simulink model "FMS"  (R2018b)
settings: configuration reference "fms_config" (kept outside this file)
values from neighbouring files (symbols this model uses):
  FMS_EXPORT = Simulink.Parameter(FMS_EXPORT_VALUE)    [fms_model_init.m]
  FMS_PARAM = Simulink.Parameter(FMS_PARAM_VALUE)    [fms_model_init.m]
undefined symbols (not defined in the file or in its folder): actuator_cmd, ax_cmd, ay_cmd, az_cmd, cmd_mask, ControlMode, ctrl_mode, DiscIntNeverNeededParam, ext_state, FMS_Cmd, FMS_CONST, home, mode, p_cmd, phi_cmd, PilotMode, psi_rate_cmd, q_cmd, r_cmd, reset, state, status, theta_cmd, throttle_cmd, timestamp, u_cmd, v_cmd, VehicleState, VehicleStatus, VTOLState, w_cmd, wp_consume, wp_current
libraries: simulink x141, FMT_Model_Lib x120, hdlsllib x13
(part 9 of 12)

== system FMS/FMS Commander/Commander/Arm/MC_Mode/Auto/Offboard/Heading_Command/Heading_Control/Error/psi_err_saturation ==
  psi_err_in : Inport
  Abs : Abs
  Compare To Constant : simulink/Logic and Bit Operations/Compare To Constant  relop=>  const=pi  OutDataTypeStr=boolean
  Constant : Constant  Value=2*pi  OutDataTypeStr=single
  Multiply : Product
  Sign : Signum
  Subtract : Sum  Inputs=-+
  Switch : Switch  Criteria=u2 > Threshold
  psi_err_rad : Outport
  wires:
  Multiply/1 -> Switch/1
  Sign/1 -> Multiply/2
  Subtract/1 -> Multiply/1
  Constant/1 -> Subtract/1
  Switch/1 -> psi_err_rad/1
  Compare To Constant/1 -> Switch/2
  Abs/1 -> Compare To Constant/1, Subtract/2
  psi_err_in/1 -> Abs/1, Switch/3, Sign/1

== system FMS/FMS Commander/Commander/Arm/MC_Mode/Auto/Offboard/Velocity_Command/Position_Control/Position_Command/Command_Mask ==
  FMS_In : Inport
  Bus Selector3 : BusSelector  OutputSignals=Auto_Cmd.cmd_mask
  Compare To Zero : simulink/Logic and Bit Operations/Compare To Zero  relop=>  OutDataTypeStr=boolean
  Mux3 : Mux  Inputs=3
  alt_cmd valid : simulink/Logic and Bit Operations/Bitwise Operator  logicop=AND  UseBitMask=on  BitMask=bin2dec('1000000000000')  BitMaskRealWorld=Stored Integer
  lat_cmd valid : simulink/Logic and Bit Operations/Bitwise Operator  logicop=AND  UseBitMask=on  BitMask=bin2dec('10000000000')  BitMaskRealWorld=Stored Integer
  lon_cmd valid : simulink/Logic and Bit Operations/Bitwise Operator  logicop=AND  UseBitMask=on  BitMask=bin2dec('100000000000')  BitMaskRealWorld=Stored Integer
  global_cmd_valid : Outport
  wires:
  Bus Selector3/1 -> alt_cmd valid/1, lat_cmd valid/1, lon_cmd valid/1  "<cmd_mask>"
  lat_cmd valid/1 -> Mux3/1
  FMS_In/1 -> Bus Selector3/1
  Mux3/1 -> Compare To Zero/1
  lon_cmd valid/1 -> Mux3/2
  alt_cmd valid/1 -> Mux3/3
  Compare To Zero/1 -> global_cmd_valid/1

== system FMS/FMS Commander/Commander/Arm/MC_Mode/Auto/Offboard/Velocity_Command/Position_Control/Position_Command/Global_Position_Command ==
  FMS_In : Inport
  Bus Selector1 : BusSelector  OutputSignals=Auto_Cmd.lat_cmd,Auto_Cmd.lon_cmd,Auto_Cmd.alt_cmd
  Bus Selector2 : BusSelector  OutputSignals=INS_Out.lat_0,INS_Out.lon_0,INS_Out.alt_0
  Constant : Constant  Value=0
  Data Type Conversion : DataTypeConversion  OutDataTypeStr=double
  Data Type Conversion1 : DataTypeConversion  OutDataTypeStr=single
  Gain : Gain  Gain=1e-7  OutDataTypeStr=double
  Gain1 : Gain  Gain=1e-7  OutDataTypeStr=double
  Gain2 : Gain  Gain=-1
  LLA2FLAT : FMT_Model_Lib/Transformation/LLA2FLAT
      settings: SourceProductName=FMT Toolbox
  Mux : Mux  Inputs=3
  Mux1 : Mux  Inputs=2
  rad2deg : Gain  Gain=180/pi  OutDataTypeStr=double
  pos_cmd_O : Outport
  wires:
  Bus Selector1/3 -> Data Type Conversion/1  "<alt_cmd>"
  Gain/1 -> Mux/1
  Mux1/1 -> rad2deg/1
  Bus Selector1/1 -> Gain/1  "<lat_cmd>"
  FMS_In/1 -> Bus Selector2/1, Bus Selector1/1
  rad2deg/1 -> LLA2FLAT/2
  Gain1/1 -> Mux/2
  Bus Selector1/2 -> Gain1/1  "<lon_cmd>"
  Mux/1 -> LLA2FLAT/1
  Bus Selector2/1 -> Mux1/1  "<lat_0>"
  Data Type Conversion/1 -> Mux/3
  Bus Selector2/2 -> Mux1/2  "<lon_0>"
  LLA2FLAT/1 -> Data Type Conversion1/1
  Data Type Conversion1/1 -> pos_cmd_O/1
  Constant/1 -> LLA2FLAT/4
  Bus Selector2/3 -> Gain2/1  "<alt_0>"
  Gain2/1 -> LLA2FLAT/3

== system FMS/FMS Commander/Commander/Arm/MC_Mode/Auto/Offboard/Velocity_Command/Position_Control/Position_Command/Local_Position_Command ==
  FMS_In : Inport
  Bus Selector4 : BusSelector  OutputSignals=Auto_Cmd.x_cmd,Auto_Cmd.y_cmd,Auto_Cmd.z_cmd
  Mux2 : Mux  Inputs=3
  pos_cmd : Outport
  wires:
  Bus Selector4/1 -> Mux2/1  "<x_cmd>"
  Bus Selector4/2 -> Mux2/2  "<y_cmd>"
  FMS_In/1 -> Bus Selector4/1
  Bus Selector4/3 -> Mux2/3  "<z_cmd>"
  Mux2/1 -> pos_cmd/1  "pos_cmd"

== system FMS/FMS Commander/Commander/Arm/MC_Mode/SubMode/Hold/Altitude Hold/Controller/Hold Control/Bus_Selection ==
  FMS_In : Inport
  Bus Selector2 : BusSelector  OutputSignals=INS_Out.h_R
  Gain : Gain  Gain=-1
  z_R_m : Outport
  wires:
  Gain/1 -> z_R_m/1
  Bus Selector2/1 -> Gain/1  "<h_R>"
  FMS_In/1 -> Bus Selector2/1

== system FMS/FMS Commander/Commander/Arm/MC_Mode/SubMode/Hold/Altitude Hold/Controller/Move Control/DeadZone ==
  u : Inport
  Dead Zone : DeadZone  LowerValue=-th  UpperValue=th  SaturateOnIntegerOverflow=on
  Gain : Gain  Gain=1/(1-th)
  y : Outport
  wires:
  Gain/1 -> y/1
  Dead Zone/1 -> Gain/1
  u/1 -> Dead Zone/1

== system FMS/FMS Commander/Commander/Arm/MC_Mode/SubMode/Hold/Altitude Hold/Controller/Move Control/TD1 ==
  v : Inport
  Integrator : DiscreteIntegrator  SampleTime=-1  ICPrevOutput=DiscIntNeverNeededParam  ICPrevScaledInput=DiscIntNeverNeededParam
  Integrator1 : DiscreteIntegrator  SampleTime=-1  ICPrevOutput=DiscIntNeverNeededParam  ICPrevScaledInput=DiscIntNeverNeededParam
  Signal Copy : SignalConversion  OverrideOpt=off
  Subtract : Sum  Inputs=+-
  "fhan " : Subsystem  mask{r0=8*9.806, h0=0.05}
      mask DialogControl ParameterGroupVar Prompt: fhan(v1,v2,r0,h0)
  v1 : Outport
  wires:
  Integrator1/1 -> Signal Copy/1, Subtract/1
  v/1 -> Subtract/2
  Integrator/1 -> "fhan "/2(v2), Integrator1/1  "v2"
  Subtract/1 -> "fhan "/1(v1)
  "fhan "/1(fhan) -> Integrator/1
  Signal Copy/1 -> v1/1

== system FMS/FMS Commander/Commander/Arm/MC_Mode/SubMode/Hold/Heading Hold/Controller/Hold Control/Bus_Selection ==
  FMS_In : Inport
  Bus Selector2 : BusSelector  OutputSignals=INS_Out.psi
  psi_rad : Outport
  wires:
  Bus Selector2/1 -> psi_rad/1  "<psi>"
  FMS_In/1 -> Bus Selector2/1

== system FMS/FMS Commander/Commander/Arm/MC_Mode/SubMode/Hold/Heading Hold/Controller/Hold Control/psi_err_saturation ==
  psi_err_in : Inport
  Abs : Abs
  Compare To Constant : simulink/Logic and Bit Operations/Compare To Constant  relop=>  const=pi  OutDataTypeStr=boolean
  Constant : Constant  Value=2*pi  OutDataTypeStr=single
  Multiply : Product
  Sign : Signum
  Subtract : Sum  Inputs=-+
  Switch : Switch  Criteria=u2 > Threshold
  psi_err_rad : Outport
  wires:
  Multiply/1 -> Switch/1
  Sign/1 -> Multiply/2
  Subtract/1 -> Multiply/1
  Constant/1 -> Subtract/1
  Switch/1 -> psi_err_rad/1
  Compare To Constant/1 -> Switch/2
  Abs/1 -> Compare To Constant/1, Subtract/2
  psi_err_in/1 -> Abs/1, Switch/3, Sign/1

== system FMS/FMS Commander/Commander/Arm/MC_Mode/SubMode/Hold/Heading Hold/Controller/Move Control/DeadZone ==
  u : Inport
  Dead Zone : DeadZone  LowerValue=-th  UpperValue=th  SaturateOnIntegerOverflow=on
  Gain : Gain  Gain=1/(1-th)
  y : Outport
  wires:
  Gain/1 -> y/1
  Dead Zone/1 -> Gain/1
  u/1 -> Dead Zone/1

== system FMS/FMS Commander/Commander/Arm/MC_Mode/SubMode/Hold/Heading Hold/Controller/Move Control/TD ==
  v : Inport
  Integrator : DiscreteIntegrator  SampleTime=-1  ICPrevOutput=DiscIntNeverNeededParam  ICPrevScaledInput=DiscIntNeverNeededParam
  Integrator1 : DiscreteIntegrator  SampleTime=-1  ICPrevOutput=DiscIntNeverNeededParam  ICPrevScaledInput=DiscIntNeverNeededParam
  Signal Copy : SignalConversion  OverrideOpt=off
  Subtract : Sum  Inputs=+-
  "fhan " : Subsystem  mask{r0=5*pi, h0=0.02}
      mask DialogControl ParameterGroupVar Prompt: fhan(v1,v2,r0,h0)
  v1 : Outport
  wires:
  "fhan "/1(fhan) -> Integrator/1
  Subtract/1 -> "fhan "/1(v1)
  Integrator/1 -> Integrator1/1, "fhan "/2(v2)  "v2"
  v/1 -> Subtract/2
  Integrator1/1 -> Subtract/1, Signal Copy/1
  Signal Copy/1 -> v1/1

== system FMS/FMS Commander/Commander/Arm/MC_Mode/SubMode/Hold/Heading Hold/Heading Control/Heading Control/Bus_Selection ==
  FMS_In : Inport
  Bus Selector2 : BusSelector  OutputSignals=INS_Out.psi
  psi_rad : Outport
  wires:
  Bus Selector2/1 -> psi_rad/1  "<psi>"
  FMS_In/1 -> Bus Selector2/1

== system FMS/FMS Commander/Commander/Arm/MC_Mode/SubMode/Hold/Heading Hold/Heading Control/Heading Control/psi_saturation ==
  psi_in : Inport
  Abs : Abs
  Add : Sum  Inputs=-+
  Compare To Constant : simulink/Logic and Bit Operations/Compare To Constant  relop=>  const=pi  OutDataTypeStr=boolean
  Constant : Constant  Value=2*pi  OutDataTypeStr=single
  Constant1 : Constant  Value=2*pi  OutDataTypeStr=single
  Multiply : Product
  Rem : Math  Operator=rem  SaturateOnIntegerOverflow=on
  Sign : Signum
  Switch : Switch  Criteria=u2 > Threshold
  psi_rad : Outport
  wires:
  Constant1/1 -> Rem/2
  psi_in/1 -> Rem/1
  Switch/1 -> psi_rad/1
  Sign/1 -> Multiply/2
  Constant/1 -> Multiply/1
  Multiply/1 -> Add/1
  Add/1 -> Switch/1
  Compare To Constant/1 -> Switch/2
  Abs/1 -> Compare To Constant/1
  Rem/1 -> Abs/1, Switch/3, Add/2, Sign/1

== system FMS/FMS Commander/Commander/Arm/MC_Mode/SubMode/Hold/Heading Hold/Heading Control/TD/fhan  ==
  v1 : Inport
  v2 : Inport  Port=2
  Abs : Abs
  Add{,1..3,5..6} (6 alike) : Sum  OutDataTypeStr=Inherit: Same as first input
  Add4 : Sum  Inputs=-++
  Divide : Product  Inputs=*/
  Gain : Gain  Gain=8
  Gain1 : Gain  Gain=0.5  OutDataTypeStr=Inherit: Same as input
  Gain2 : Gain  Gain=0.5  OutDataTypeStr=Inherit: Same as input
  Gain3 : Gain  Gain=0.5  OutDataTypeStr=Inherit: Same as input
  Gain4 : Gain  Gain=-1  OutDataTypeStr=Inherit: Same as input
  Multiply{,1..3} (4 alike) : Product  OutDataTypeStr=Inherit: Same as first input
  Multiply4 : Product  OutDataTypeStr=single
  Multiply5 : Product  Inputs=3
  Multiply6 : Product  OutDataTypeStr=single
  Sign{,1..6} (7 alike) : Signum
  Sqrt : Sqrt  SaturateOnIntegerOverflow=on
  Square : Math  Operator=square  SaturateOnIntegerOverflow=on
  Subtract{,1..5} (6 alike) : Sum  Inputs=+-  OutDataTypeStr=Inherit: Same as first input
  Subtract6 : Sum  Inputs=-+  OutDataTypeStr=Inherit: Same as first input
  const : Constant  Value=r0  OutDataTypeStr=single
  const1 : Constant  Value=h0  OutDataTypeStr=single
  fhan : Outport
  wires:
  Sign1/1 -> Subtract2/1
  Multiply2/1 -> Sqrt/1
  Square/1 -> Multiply/2
  Gain1/1 -> Multiply3/2
  Multiply6/1 -> Subtract6/1
  Multiply/1 -> Multiply2/2, Add1/1, Add3/2, Subtract1/2, Add6/2, Subtract3/2, Divide/2, Subtract/2  "d"
  Add6/1 -> Sign3/1
  Sign3/1 -> Subtract4/1
  Sign6/1 -> Multiply6/1
  Multiply5/1 -> Subtract6/2
  Gain4/1 -> Multiply5/1
  Subtract4/1 -> Gain3/1
  Add2/1 -> Add5/1, Add4/1  "a2"
  Subtract2/1 -> Gain2/1
  Add/1 -> Abs/1, Sign/1, Add4/2, Add3/1, Subtract1/1  "y"
  Multiply1/1 -> Add/2, Add2/2, Add4/3  "a0"
  Add5/1 -> Add6/1, Subtract3/1, Divide/1, Sign5/1, Sign6/1  "a"
  const1/1 -> Square/1, Multiply1/2
  Multiply4/1 -> Add5/2
  Subtract5/1 -> Multiply5/2
  Add3/1 -> Sign1/1
  const/1 -> Multiply/1, Gain4/1, Multiply6/2
  Gain/1 -> Add1/2
  Multiply3/1 -> Add2/1
  Divide/1 -> Subtract5/1
  Subtract1/1 -> Sign2/1
  Add1/1 -> Multiply2/1
  Subtract3/1 -> Sign4/1
  Sqrt/1 -> Subtract/1  "a1"
  Sign5/1 -> Subtract5/2
  Add4/1 -> Multiply4/1
  Abs/1 -> Gain/1
  Sign4/1 -> Subtract4/2
  Sign2/1 -> Subtract2/2
  Subtract6/1 -> fhan/1
  Subtract/1 -> Gain1/1
  Gain3/1 -> Multiply5/3  "sa"
  v2/1 -> Multiply1/1
  Gain2/1 -> Multiply4/2  "sy"
  Sign/1 -> Multiply3/1
  v1/1 -> Add/1

== system FMS/FMS Commander/Commander/Arm/MC_Mode/SubMode/Hold/Position Hold/Controller/Hold Control/Bus_Selection ==
  FMS_In : Inport
  Bus Selector2 : BusSelector  OutputSignals=INS_Out.x_R,INS_Out.y_R
  Mux : Mux  Inputs=2
  xy_R_O_m : Outport
  wires:
  Bus Selector2/2 -> Mux/2  "<y_R>"
  Mux/1 -> xy_R_O_m/1
  Bus Selector2/1 -> Mux/1  "<x_R>"
  FMS_In/1 -> Bus Selector2/1

== system FMS/FMS Commander/Commander/Arm/MC_Mode/SubMode/Hold/Position Hold/Controller/Move Control/DeadZone ==
  u : Inport
  Dead Zone : DeadZone  LowerValue=-th  UpperValue=th  SaturateOnIntegerOverflow=on
  Gain : Gain  Gain=1/(1-th)
  y : Outport
  wires:
  Gain/1 -> y/1
  Dead Zone/1 -> Gain/1
  u/1 -> Dead Zone/1

== system FMS/FMS Commander/Commander/Arm/MC_Mode/SubMode/Hold/Position Hold/Controller/Move Control/DeadZone1 ==
  u : Inport
  Dead Zone : DeadZone  LowerValue=-th  UpperValue=th  SaturateOnIntegerOverflow=on
  Gain : Gain  Gain=1/(1-th)
  y : Outport
  wires:
  u/1 -> Dead Zone/1
  Dead Zone/1 -> Gain/1
  Gain/1 -> y/1

== system FMS/FMS Commander/Commander/Arm/MC_Mode/SubMode/Hold/Position Hold/Controller/Move Control/TD ==
  v : Inport
  Integrator : DiscreteIntegrator  SampleTime=-1  ICPrevOutput=DiscIntNeverNeededParam  ICPrevScaledInput=DiscIntNeverNeededParam
  Integrator1 : DiscreteIntegrator  SampleTime=-1  ICPrevOutput=DiscIntNeverNeededParam  ICPrevScaledInput=DiscIntNeverNeededParam
  Signal Copy : SignalConversion  OverrideOpt=off
  Subtract : Sum  Inputs=+-
  "fhan " : Subsystem  mask{r0=6*9.806, h0=0.05}
      mask DialogControl ParameterGroupVar Prompt: fhan(v1,v2,r0,h0)
  v1 : Outport
  wires:
  "fhan "/1(fhan) -> Integrator/1
  Subtract/1 -> "fhan "/1(v1)
  Integrator/1 -> Integrator1/1, "fhan "/2(v2)  "v2"
  v/1 -> Subtract/2
  Integrator1/1 -> Subtract/1, Signal Copy/1
  Signal Copy/1 -> v1/1

== system FMS/FMS Commander/Commander/Arm/MC_Mode/SubMode/Return/Heading Commander/Heading Control/Heading Control/Bus_Selection ==
  FMS_In : Inport
  Bus Selector2 : BusSelector  OutputSignals=INS_Out.psi
  psi_rad : Outport
  wires:
  Bus Selector2/1 -> psi_rad/1  "<psi>"
  FMS_In/1 -> Bus Selector2/1

== system FMS/FMS Commander/Commander/Arm/MC_Mode/SubMode/Return/Heading Commander/Heading Control/Heading Control/psi_saturation ==
  psi_in : Inport
  Abs : Abs
  Add : Sum  Inputs=-+
  Compare To Constant : simulink/Logic and Bit Operations/Compare To Constant  relop=>  const=pi  OutDataTypeStr=boolean
  Constant : Constant  Value=2*pi  OutDataTypeStr=single
  Constant1 : Constant  Value=2*pi  OutDataTypeStr=single
  Multiply : Product
  Rem : Math  Operator=rem  SaturateOnIntegerOverflow=on
  Sign : Signum
  Switch : Switch  Criteria=u2 > Threshold
  psi_rad : Outport
  wires:
  Constant1/1 -> Rem/2
  psi_in/1 -> Rem/1
  Switch/1 -> psi_rad/1
  Sign/1 -> Multiply/2
  Constant/1 -> Multiply/1
  Multiply/1 -> Add/1
  Add/1 -> Switch/1
  Compare To Constant/1 -> Switch/2
  Abs/1 -> Compare To Constant/1
  Rem/1 -> Abs/1, Switch/3, Add/2, Sign/1

== system FMS/FMS Commander/Commander/Arm/MC_Mode/SubMode/Return/Heading Commander/Heading Control/TD/fhan  ==
  v1 : Inport
  v2 : Inport  Port=2
  Abs : Abs
  Add{,1..3,5..6} (6 alike) : Sum  OutDataTypeStr=Inherit: Same as first input
  Add4 : Sum  Inputs=-++
  Divide : Product  Inputs=*/
  Gain : Gain  Gain=8
  Gain1 : Gain  Gain=0.5  OutDataTypeStr=Inherit: Same as input
  Gain2 : Gain  Gain=0.5  OutDataTypeStr=Inherit: Same as input
  Gain3 : Gain  Gain=0.5  OutDataTypeStr=Inherit: Same as input
  Gain4 : Gain  Gain=-1  OutDataTypeStr=Inherit: Same as input
  Multiply{,1..3} (4 alike) : Product  OutDataTypeStr=Inherit: Same as first input
  Multiply4 : Product  OutDataTypeStr=single
  Multiply5 : Product  Inputs=3
  Multiply6 : Product  OutDataTypeStr=single
  Sign{,1..6} (7 alike) : Signum
  Sqrt : Sqrt  SaturateOnIntegerOverflow=on
  Square : Math  Operator=square  SaturateOnIntegerOverflow=on
  Subtract{,1..5} (6 alike) : Sum  Inputs=+-  OutDataTypeStr=Inherit: Same as first input
  Subtract6 : Sum  Inputs=-+  OutDataTypeStr=Inherit: Same as first input
  const : Constant  Value=r0  OutDataTypeStr=single
  const1 : Constant  Value=h0  OutDataTypeStr=single
  fhan : Outport
  wires:
  Sign1/1 -> Subtract2/1
  Multiply2/1 -> Sqrt/1
  Square/1 -> Multiply/2
  Gain1/1 -> Multiply3/2
  Multiply6/1 -> Subtract6/1
  Multiply/1 -> Multiply2/2, Add1/1, Add3/2, Subtract1/2, Add6/2, Subtract3/2, Divide/2, Subtract/2  "d"
  Add6/1 -> Sign3/1
  Sign3/1 -> Subtract4/1
  Sign6/1 -> Multiply6/1
  Multiply5/1 -> Subtract6/2
  Gain4/1 -> Multiply5/1
  Subtract4/1 -> Gain3/1
  Add2/1 -> Add5/1, Add4/1  "a2"
  Subtract2/1 -> Gain2/1
  Add/1 -> Abs/1, Sign/1, Add4/2, Add3/1, Subtract1/1  "y"
  Multiply1/1 -> Add/2, Add2/2, Add4/3  "a0"
  Add5/1 -> Add6/1, Subtract3/1, Divide/1, Sign5/1, Sign6/1  "a"
  const1/1 -> Square/1, Multiply1/2
  Multiply4/1 -> Add5/2
  Subtract5/1 -> Multiply5/2
  Add3/1 -> Sign1/1
  const/1 -> Multiply/1, Gain4/1, Multiply6/2
  Gain/1 -> Add1/2
  Multiply3/1 -> Add2/1
  Divide/1 -> Subtract5/1
  Subtract1/1 -> Sign2/1
  Add1/1 -> Multiply2/1
  Subtract3/1 -> Sign4/1
  Sqrt/1 -> Subtract/1  "a1"
  Sign5/1 -> Subtract5/2
  Add4/1 -> Multiply4/1
  Abs/1 -> Gain/1
  Sign4/1 -> Subtract4/2
  Sign2/1 -> Subtract2/2
  Subtract6/1 -> fhan/1
  Subtract/1 -> Gain1/1
  Gain3/1 -> Multiply5/3  "sa"
  v2/1 -> Multiply1/1
  Gain2/1 -> Multiply4/2  "sy"
  Sign/1 -> Multiply3/1
  v1/1 -> Add/1

== system FMS/FMS Commander/Commander/Arm/MC_Mode/SubMode/Return/Velocity Commander/Hold Position/Altitude Hold/Controller ==
  motion_state : Inport
  In Bus Element : Inport  Port=2  PortName=FMS_In
  In Bus Element1 : Inport  Port=2  PortName=FMS_In
  Brake Control : Subsystem  TreatAsAtomicUnit=on
  Hold Control : Subsystem  TreatAsAtomicUnit=on
  Merge : Merge  Inputs=3
  Move Control : Subsystem  TreatAsAtomicUnit=on
  Saturation1 : Saturate  UpperLimit=FMS_PARAM.VEL_Z_LIM  LowerLimit=-FMS_PARAM.VEL_Z_LIM
  Switch Case : SwitchCase  CaseConditions={MotionState.Hold, MotionState.Brake, MotionState.Move}  ShowDefaultCase=off
  w_cmd_mPs : Outport
  wires:
  Move Control/1(w_cmd_mPs) -> Merge/3
  Brake Control/1(psi_rate_cmd_radPs) -> Merge/2
  Hold Control/1(w_cmd_mPs) -> Merge/1
  In Bus Element/1 -> Hold Control/1(FMS_In)
  Switch Case/3 -> Move Control/Action
  Switch Case/2 -> Brake Control/Action
  Switch Case/1 -> Hold Control/Action
  motion_state/1 -> Switch Case/1
  Saturation1/1 -> w_cmd_mPs/1
  Merge/1 -> Saturation1/1
  In Bus Element1/1 -> Move Control/1(FMS_In)

== system FMS/FMS Commander/Commander/Arm/MC_Mode/SubMode/Return/Velocity Commander/Hold Position/Altitude Hold/Detect Movement ==
  FMS_In : Inport
  Abs : Abs
  Bus Selector : BusSelector  OutputSignals=INS_Out.vd
  Constant : Constant  Value=0  OutDataTypeStr=Inherit: Inherit via back propagation
  Motion Status : Stateflow chart  TreatAsAtomicUnit=on
  motion_state : Outport
  wires:
  FMS_In/1 -> Bus Selector/1
  Motion Status/1(state) -> motion_state/1
  Constant/1 -> Motion Status/1(motion_req)
  Abs/1 -> Motion Status/2(speed)
  Bus Selector/1 -> Abs/1  "<vd>"

== system FMS/FMS Commander/Commander/Arm/MC_Mode/SubMode/Return/Velocity Commander/Hold Position/Position Hold/Controller ==
  motion_state : Inport
  In Bus Element : Inport  Port=2  PortName=FMS_In
  In Bus Element1 : Inport  Port=2  PortName=FMS_In
  Brake Control : Subsystem  TreatAsAtomicUnit=on
  Hold Control : Subsystem  TreatAsAtomicUnit=on
  Merge : Merge  Inputs=3
  Move Control : Subsystem  TreatAsAtomicUnit=on
  Saturation1 : Saturate  UpperLimit=FMS_PARAM.VEL_XY_LIM  LowerLimit=-FMS_PARAM.VEL_XY_LIM
  Switch Case : SwitchCase  CaseConditions={MotionState.Hold, MotionState.Brake, MotionState.Move}  ShowDefaultCase=off
  uv_cmd_mPs : Outport
  wires:
  Move Control/1(uv_cmd_mPs) -> Merge/3
  Brake Control/1(uv_cmd_mPs) -> Merge/2
  Hold Control/1(uv_cmd_mPs) -> Merge/1
  In Bus Element/1 -> Hold Control/1(FMS_In)
  Switch Case/3 -> Move Control/Action
  Switch Case/2 -> Brake Control/Action
  Switch Case/1 -> Hold Control/Action
  motion_state/1 -> Switch Case/1
  Saturation1/1 -> uv_cmd_mPs/1
  Merge/1 -> Saturation1/1
  In Bus Element1/1 -> Move Control/1(FMS_In)

== system FMS/FMS Commander/Commander/Arm/MC_Mode/SubMode/Return/Velocity Commander/Hold Position/Position Hold/Detect Movement ==
  FMS_In : Inport
  Add : Sum
  Bus Selector1 : BusSelector  OutputSignals=INS_Out.vn,INS_Out.ve
  Constant : Constant  Value=0  OutDataTypeStr=Inherit: Inherit via back propagation
  Motion State : Stateflow chart  TreatAsAtomicUnit=on
  Sqrt : Sqrt  SaturateOnIntegerOverflow=on
  Square : Math  Operator=square  SaturateOnIntegerOverflow=on
  Square1 : Math  Operator=square  SaturateOnIntegerOverflow=on
  motion_state : Outport
  wires:
  FMS_In/1 -> Bus Selector1/1
  Add/1 -> Sqrt/1
  Square1/1 -> Add/2
  Square/1 -> Add/1
  Motion State/1(state) -> motion_state/1  "pos_ms"
  Sqrt/1 -> Motion State/2(speed)
  Bus Selector1/1 -> Square/1  "<vn>"
  Bus Selector1/2 -> Square1/1  "<ve>"
  Constant/1 -> Motion State/1(motion_req)

== system FMS/FMS Commander/Commander/Arm/FW_Mode/Assist/Altitude/Altitude Command/Controller/Move Control/TD1/fhan  ==
  v1 : Inport
  v2 : Inport  Port=2
  Abs : Abs
  Add{,1..3,5..6} (6 alike) : Sum  OutDataTypeStr=Inherit: Same as first input
  Add4 : Sum  Inputs=-++
  Divide : Product  Inputs=*/
  Gain : Gain  Gain=8
  Gain1 : Gain  Gain=0.5  OutDataTypeStr=Inherit: Same as input
  Gain2 : Gain  Gain=0.5  OutDataTypeStr=Inherit: Same as input
  Gain3 : Gain  Gain=0.5  OutDataTypeStr=Inherit: Same as input
  Gain4 : Gain  Gain=-1  OutDataTypeStr=Inherit: Same as input
  Multiply{,1..3} (4 alike) : Product  OutDataTypeStr=Inherit: Same as first input
  Multiply4 : Product  OutDataTypeStr=single
  Multiply5 : Product  Inputs=3
  Multiply6 : Product  OutDataTypeStr=single
  Sign{,1..6} (7 alike) : Signum
  Sqrt : Sqrt  SaturateOnIntegerOverflow=on
  Square : Math  Operator=square  SaturateOnIntegerOverflow=on
  Subtract{,1..5} (6 alike) : Sum  Inputs=+-  OutDataTypeStr=Inherit: Same as first input
  Subtract6 : Sum  Inputs=-+  OutDataTypeStr=Inherit: Same as first input
  const : Constant  Value=r0  OutDataTypeStr=single
  const1 : Constant  Value=h0  OutDataTypeStr=single
  fhan : Outport
  wires:
  Sign1/1 -> Subtract2/1
  Multiply2/1 -> Sqrt/1
  Square/1 -> Multiply/2
  Gain1/1 -> Multiply3/2
  Multiply6/1 -> Subtract6/1
  Multiply/1 -> Multiply2/2, Add1/1, Add3/2, Subtract1/2, Add6/2, Subtract3/2, Divide/2, Subtract/2  "d"
  Add6/1 -> Sign3/1
  Sign3/1 -> Subtract4/1
  Sign6/1 -> Multiply6/1
  Multiply5/1 -> Subtract6/2
  Gain4/1 -> Multiply5/1
  Subtract4/1 -> Gain3/1
  Add2/1 -> Add5/1, Add4/1  "a2"
  Subtract2/1 -> Gain2/1
  Add/1 -> Abs/1, Sign/1, Add4/2, Add3/1, Subtract1/1  "y"
  Multiply1/1 -> Add/2, Add2/2, Add4/3  "a0"
  Add5/1 -> Add6/1, Subtract3/1, Divide/1, Sign5/1, Sign6/1  "a"
  const1/1 -> Square/1, Multiply1/2
  Multiply4/1 -> Add5/2
  Subtract5/1 -> Multiply5/2
  Add3/1 -> Sign1/1
  const/1 -> Multiply/1, Gain4/1, Multiply6/2
  Gain/1 -> Add1/2
  Multiply3/1 -> Add2/1
  Divide/1 -> Subtract5/1
  Subtract1/1 -> Sign2/1
  Add1/1 -> Multiply2/1
  Subtract3/1 -> Sign4/1
  Sqrt/1 -> Subtract/1  "a1"
  Sign5/1 -> Subtract5/2
  Add4/1 -> Multiply4/1
  Abs/1 -> Gain/1
  Sign4/1 -> Subtract4/2
  Sign2/1 -> Subtract2/2
  Subtract6/1 -> fhan/1
  Subtract/1 -> Gain1/1
  Gain3/1 -> Multiply5/3  "sa"
  v2/1 -> Multiply1/1
  Gain2/1 -> Multiply4/2  "sy"
  Sign/1 -> Multiply3/1
  v1/1 -> Add/1

== system FMS/FMS Commander/Commander/Arm/FW_Mode/Assist/Position/Altitude Command/Controller/Move Control/TD1/fhan  ==
  v1 : Inport
  v2 : Inport  Port=2
  Abs : Abs
  Add{,1..3,5..6} (6 alike) : Sum  OutDataTypeStr=Inherit: Same as first input
  Add4 : Sum  Inputs=-++
  Divide : Product  Inputs=*/
  Gain : Gain  Gain=8
  Gain1 : Gain  Gain=0.5  OutDataTypeStr=Inherit: Same as input
  Gain2 : Gain  Gain=0.5  OutDataTypeStr=Inherit: Same as input
  Gain3 : Gain  Gain=0.5  OutDataTypeStr=Inherit: Same as input
  Gain4 : Gain  Gain=-1  OutDataTypeStr=Inherit: Same as input
  Multiply{,1..3} (4 alike) : Product  OutDataTypeStr=Inherit: Same as first input
  Multiply4 : Product  OutDataTypeStr=single
  Multiply5 : Product  Inputs=3
  Multiply6 : Product  OutDataTypeStr=single
  Sign{,1..6} (7 alike) : Signum
  Sqrt : Sqrt  SaturateOnIntegerOverflow=on
  Square : Math  Operator=square  SaturateOnIntegerOverflow=on
  Subtract{,1..5} (6 alike) : Sum  Inputs=+-  OutDataTypeStr=Inherit: Same as first input
  Subtract6 : Sum  Inputs=-+  OutDataTypeStr=Inherit: Same as first input
  const : Constant  Value=r0  OutDataTypeStr=single
  const1 : Constant  Value=h0  OutDataTypeStr=single
  fhan : Outport
  wires:
  Sign1/1 -> Subtract2/1
  Multiply2/1 -> Sqrt/1
  Square/1 -> Multiply/2
  Gain1/1 -> Multiply3/2
  Multiply6/1 -> Subtract6/1
  Multiply/1 -> Multiply2/2, Add1/1, Add3/2, Subtract1/2, Add6/2, Subtract3/2, Divide/2, Subtract/2  "d"
  Add6/1 -> Sign3/1
  Sign3/1 -> Subtract4/1
  Sign6/1 -> Multiply6/1
  Multiply5/1 -> Subtract6/2
  Gain4/1 -> Multiply5/1
  Subtract4/1 -> Gain3/1
  Add2/1 -> Add5/1, Add4/1  "a2"
  Subtract2/1 -> Gain2/1
  Add/1 -> Abs/1, Sign/1, Add4/2, Add3/1, Subtract1/1  "y"
  Multiply1/1 -> Add/2, Add2/2, Add4/3  "a0"
  Add5/1 -> Add6/1, Subtract3/1, Divide/1, Sign5/1, Sign6/1  "a"
  const1/1 -> Square/1, Multiply1/2
  Multiply4/1 -> Add5/2
  Subtract5/1 -> Multiply5/2
  Add3/1 -> Sign1/1
  const/1 -> Multiply/1, Gain4/1, Multiply6/2
  Gain/1 -> Add1/2
  Multiply3/1 -> Add2/1
  Divide/1 -> Subtract5/1
  Subtract1/1 -> Sign2/1
  Add1/1 -> Multiply2/1
  Subtract3/1 -> Sign4/1
  Sqrt/1 -> Subtract/1  "a1"
  Sign5/1 -> Subtract5/2
  Add4/1 -> Multiply4/1
  Abs/1 -> Gain/1
  Sign4/1 -> Subtract4/2
  Sign2/1 -> Subtract2/2
  Subtract6/1 -> fhan/1
  Subtract/1 -> Gain1/1
  Gain3/1 -> Multiply5/3  "sa"
  v2/1 -> Multiply1/1
  Gain2/1 -> Multiply4/2  "sy"
  Sign/1 -> Multiply3/1
  v1/1 -> Add/1

== system FMS/FMS Commander/Commander/Arm/FW_Mode/Assist/Position/Position Command/Controller/Hold Control/Lateral_Acceleration/L1_Lateral_Acceleration ==
  L1 : Inport
  Vg : Inport  Port=2
  l1_path : Inport  Port=3
  Constant : Constant  Value=0.5  OutDataTypeStr=Inherit: Inherit via back propagation
  Divide : Product  Inputs=*/
  Gain : Gain  Gain=2
  Included Angle : Subsystem
  Max : MinMax  Function=max  Inputs=2
  Min : MinMax  Inputs=2
  Multiply1 : Product
  Saturation : Saturate  UpperLimit=pi/2  LowerLimit=-pi/2
  Sin : Trigonometry
  Square : Math  Operator=square  SaturateOnIntegerOverflow=on
  Vector Modulus : FMT_Model_Lib/Math/Vector Modulus
      settings: SourceProductName=FMT Toolbox
  Vector Modulus1 : FMT_Model_Lib/Math/Vector Modulus
      settings: SourceProductName=FMT Toolbox
  Vector Normalize : FMT_Model_Lib/Math/Vector Normalize
      settings: SourceProductName=FMT Toolbox
  Vector Normalize1 : FMT_Model_Lib/Math/Vector Normalize
      settings: SourceProductName=FMT Toolbox
  l1_a_cmd : Outport
  wires:
  Vector Normalize/1 -> Included Angle/1(vec1)
  Included Angle/1(angle_rad) -> Saturation/1  "L1_alpha"
  L1/1 -> Min/1
  Multiply1/1 -> Divide/1
  Divide/1 -> l1_a_cmd/1  "l1_a_cmd"
  Vector Normalize1/1 -> Included Angle/2(vec2)
  Sin/1 -> Multiply1/1  "sin_alpha"
  l1_path/1 -> Vector Modulus1/1, Vector Normalize1/1
  Saturation/1 -> Sin/1
  Vg/1 -> Vector Normalize/1, Vector Modulus/1
  Square/1 -> Gain/1
  Gain/1 -> Multiply1/2
  Min/1 -> Divide/2
  Max/1 -> Min/2
  Vector Modulus/1 -> Square/1
  Vector Modulus1/1 -> Max/1
  Constant/1 -> Max/2

== system FMS/FMS Commander/Commander/Arm/FW_Mode/Assist/Position/Position Command/Controller/Hold Control/Velocity_Controller/Error ==
  INS_Out : Inport
  Bus_Select : Subsystem
  Constant : Constant  Value=0  OutDataTypeStr=single
  Sum : Sum  Inputs=|+-
  v_err_C_mPs : Outport
  wires:
  Sum/1 -> v_err_C_mPs/1  "v_error_C_mPs"
  INS_Out/1 -> Bus_Select/1(INS_Out)
  Bus_Select/1(v_est_C_mPs) -> Sum/2  "v_est_C_mPs"
  Constant/1 -> Sum/1

== system FMS/FMS Commander/Commander/Arm/FW_Mode/Assist/Position/Position Command/Controller/Hold Control/Velocity_Controller/PID_Controller ==
  uv_err_C_mPs : Inport
  reset : Inport  Port=2
  Add : Sum  Inputs=+++
  D_Control : Subsystem  mask{kd=0, max_d=1, min_d=-1}
  I_Control : Subsystem  mask{ki=0.5, max_i=1, min_i=-1}
  P_Control : Subsystem  mask{kp=1.2}
  accel_cmd_C : Outport
  wires:
  uv_err_C_mPs/1 -> P_Control/1(err), I_Control/1(err), D_Control/1(err)
  reset/1 -> I_Control/2(reset), D_Control/2(reset)
  P_Control/1(p_out) -> Add/1  "accel_p_out"
  I_Control/1(i_out) -> Add/2  "accel_i_out"
  D_Control/1(d_out) -> Add/3  "accel_d_out"
  Add/1 -> accel_cmd_C/1

== system FMS/FMS Commander/Commander/Arm/FW_Mode/Assist/Position/Position Command/Controller/Move Control/TD/fhan  ==
  v1 : Inport
  v2 : Inport  Port=2
  Abs : Abs
  Add{,1..3,5..6} (6 alike) : Sum  OutDataTypeStr=Inherit: Same as first input
  Add4 : Sum  Inputs=-++
  Divide : Product  Inputs=*/
  Gain : Gain  Gain=8
  Gain1 : Gain  Gain=0.5  OutDataTypeStr=Inherit: Same as input
  Gain2 : Gain  Gain=0.5  OutDataTypeStr=Inherit: Same as input
  Gain3 : Gain  Gain=0.5  OutDataTypeStr=Inherit: Same as input
  Gain4 : Gain  Gain=-1  OutDataTypeStr=Inherit: Same as input
  Multiply{,1..3} (4 alike) : Product  OutDataTypeStr=Inherit: Same as first input
  Multiply4 : Product  OutDataTypeStr=single
  Multiply5 : Product  Inputs=3
  Multiply6 : Product  OutDataTypeStr=single
  Sign{,1..6} (7 alike) : Signum
  Sqrt : Sqrt  SaturateOnIntegerOverflow=on
  Square : Math  Operator=square  SaturateOnIntegerOverflow=on
  Subtract{,1..5} (6 alike) : Sum  Inputs=+-  OutDataTypeStr=Inherit: Same as first input
  Subtract6 : Sum  Inputs=-+  OutDataTypeStr=Inherit: Same as first input
  const : Constant  Value=r0  OutDataTypeStr=single
  const1 : Constant  Value=h0  OutDataTypeStr=single
  fhan : Outport
  wires:
  v1/1 -> Add/1
  Sign/1 -> Multiply3/1
  Gain2/1 -> Multiply4/2  "sy"
  v2/1 -> Multiply1/1
  Gain3/1 -> Multiply5/3  "sa"
  Subtract/1 -> Gain1/1
  Subtract6/1 -> fhan/1
  Sign2/1 -> Subtract2/2
  Sign4/1 -> Subtract4/2
  Abs/1 -> Gain/1
  Add4/1 -> Multiply4/1
  Sign5/1 -> Subtract5/2
  Sqrt/1 -> Subtract/1  "a1"
  Subtract3/1 -> Sign4/1
  Add1/1 -> Multiply2/1
  Subtract1/1 -> Sign2/1
  Divide/1 -> Subtract5/1
  Multiply3/1 -> Add2/1
  Gain/1 -> Add1/2
  const/1 -> Multiply6/2, Gain4/1, Multiply/1
  Add3/1 -> Sign1/1
  Subtract5/1 -> Multiply5/2
  Multiply4/1 -> Add5/2
  const1/1 -> Multiply1/2, Square/1
  Add5/1 -> Sign6/1, Sign5/1, Divide/1, Subtract3/1, Add6/1  "a"
  Multiply1/1 -> Add4/3, Add2/2, Add/2  "a0"
  Add/1 -> Subtract1/1, Add3/1, Add4/2, Sign/1, Abs/1  "y"
  Subtract2/1 -> Gain2/1
  Add2/1 -> Add4/1, Add5/1  "a2"
  Subtract4/1 -> Gain3/1
  Gain4/1 -> Multiply5/1
  Multiply5/1 -> Subtract6/2
  Sign6/1 -> Multiply6/1
  Sign3/1 -> Subtract4/1
  Add6/1 -> Sign3/1
  Multiply/1 -> Subtract/2, Divide/2, Subtract3/2, Add6/2, Subtract1/2, Add3/2, Add1/1, Multiply2/2  "d"
  Multiply6/1 -> Subtract6/1
  Gain1/1 -> Multiply3/2
  Square/1 -> Multiply/2
  Multiply2/1 -> Sqrt/1
  Sign1/1 -> Subtract2/1

== system FMS/FMS Commander/Commander/Arm/FW_Mode/Auto/Mission/Mission_SubSystem/Position Command/L1 Control/L1_Core/L1_Lateral_Acceleration ==
  L1 : Inport
  Vg : Inport  Port=2
  l1_path : Inport  Port=3
  Divide : Product  Inputs=*/
  Gain : Gain  Gain=2
  Included Angle : Subsystem
  Multiply1 : Product
  Saturation : Saturate  UpperLimit=pi/2  LowerLimit=-pi/2
  Sin : Trigonometry
  Square : Math  Operator=square  SaturateOnIntegerOverflow=on
  Vector Modulus : FMT_Model_Lib/Math/Vector Modulus
      settings: SourceProductName=FMT Toolbox
  Vector Normalize : FMT_Model_Lib/Math/Vector Normalize
      settings: SourceProductName=FMT Toolbox
  Vector Normalize1 : FMT_Model_Lib/Math/Vector Normalize
      settings: SourceProductName=FMT Toolbox
  l1_a_cmd : Outport
  wires:
  Vector Normalize/1 -> Included Angle/1(vec1)
  Included Angle/1(angle_rad) -> Saturation/1  "L1_alpha"
  Multiply1/1 -> Divide/1
  Divide/1 -> l1_a_cmd/1  "l1_a_cmd"
  Vector Normalize1/1 -> Included Angle/2(vec2)
  Sin/1 -> Multiply1/1  "sin_alpha"
  l1_path/1 -> Vector Normalize1/1
  Saturation/1 -> Sin/1
  Vg/1 -> Vector Normalize/1, Vector Modulus/1
  Square/1 -> Gain/1
  Gain/1 -> Multiply1/2
  L1/1 -> Divide/2
  Vector Modulus/1 -> Square/1

== system FMS/FMS Commander/Commander/Arm/FW_Mode/SubMode/Return/Position Command/L1 Control/L1_Core/L1_Lateral_Acceleration/Included Angle ==
  vec1 : Inport
  vec2 : Inport  Port=2
  2D Cross Product : FMT_Model_Lib/Math/2D Cross Product
      settings: SourceProductName=FMT Toolbox
  Acos : Trigonometry  Operator=acos
  Constant4 : Constant  OutDataTypeStr=single
  Demux : Demux  Outputs=2
  Demux1 : Demux  Outputs=2
  Dot Product : DotProduct  InputSameDT=on  OutDataTypeStr=Inherit: Inherit via internal rule
  Multiply : Product
  Mux : Mux  Inputs=2
  Mux1 : Mux  Inputs=2
  Sign1 : Signum
  Switch2 : Switch  Criteria=u2 ~= 0
  Vector Normalize : FMT_Model_Lib/Math/Vector Normalize
      settings: SourceProductName=FMT Toolbox
  Vector Normalize1 : FMT_Model_Lib/Math/Vector Normalize
      settings: SourceProductName=FMT Toolbox
  angle_rad : Outport
  wires:
  Switch2/1 -> Multiply/2
  Acos/1 -> Multiply/1
  Mux/1 -> Vector Normalize1/1
  vec2/1 -> Demux/1
  Constant4/1 -> Switch2/3
  Demux/1 -> Mux/2
  vec1/1 -> Demux1/1
  Multiply/1 -> angle_rad/1
  2D Cross Product/1 -> Sign1/1
  Vector Normalize/1 -> 2D Cross Product/2, Dot Product/1
  Demux/2 -> Mux/1
  Vector Normalize1/1 -> 2D Cross Product/1, Dot Product/2
  Sign1/1 -> Switch2/2, Switch2/1
  Demux1/2 -> Mux1/1
  Mux1/1 -> Vector Normalize/1
  Demux1/1 -> Mux1/2
  Dot Product/1 -> Acos/1

== system FMS/FMS Commander/Commander/Arm/FW_Mode/SubMode/Takeoff/Position Command/L1 Control/L1_Core/L1_Lateral_Acceleration/Included Angle ==
  vec1 : Inport
  vec2 : Inport  Port=2
  2D Cross Product : FMT_Model_Lib/Math/2D Cross Product
      settings: SourceProductName=FMT Toolbox
  Acos : Trigonometry  Operator=acos
  Constant4 : Constant  OutDataTypeStr=single
  Demux : Demux  Outputs=2
  Demux1 : Demux  Outputs=2
  Dot Product : DotProduct  InputSameDT=on  OutDataTypeStr=Inherit: Inherit via internal rule
  Multiply : Product
  Mux : Mux  Inputs=2
  Mux1 : Mux  Inputs=2
  Sign1 : Signum
  Switch2 : Switch  Criteria=u2 ~= 0
  Vector Normalize : FMT_Model_Lib/Math/Vector Normalize
      settings: SourceProductName=FMT Toolbox
  Vector Normalize1 : FMT_Model_Lib/Math/Vector Normalize
      settings: SourceProductName=FMT Toolbox
  angle_rad : Outport
  wires:
  Switch2/1 -> Multiply/2
  Acos/1 -> Multiply/1
  Mux/1 -> Vector Normalize1/1
  vec2/1 -> Demux/1
  Constant4/1 -> Switch2/3
  Demux/1 -> Mux/2
  vec1/1 -> Demux1/1
  Multiply/1 -> angle_rad/1
  2D Cross Product/1 -> Sign1/1
  Vector Normalize/1 -> 2D Cross Product/2, Dot Product/1
  Demux/2 -> Mux/1
  Vector Normalize1/1 -> 2D Cross Product/1, Dot Product/2
  Sign1/1 -> Switch2/2, Switch2/1
  Demux1/2 -> Mux1/1
  Mux1/1 -> Vector Normalize/1
  Demux1/1 -> Mux1/2
  Dot Product/1 -> Acos/1

== system FMS/FMS Commander/Commander/Arm/MC_Mode/Assist/Altitude/Heading Command/Controller/Move Control/TD/fhan  ==
  v1 : Inport
  v2 : Inport  Port=2
  Abs : Abs
  Add{,1..3,5..6} (6 alike) : Sum  OutDataTypeStr=Inherit: Same as first input
  Add4 : Sum  Inputs=-++
  Divide : Product  Inputs=*/
  Gain : Gain  Gain=8
  Gain1 : Gain  Gain=0.5  OutDataTypeStr=Inherit: Same as input
  Gain2 : Gain  Gain=0.5  OutDataTypeStr=Inherit: Same as input
  Gain3 : Gain  Gain=0.5  OutDataTypeStr=Inherit: Same as input
  Gain4 : Gain  Gain=-1  OutDataTypeStr=Inherit: Same as input
  Multiply{,1..3} (4 alike) : Product  OutDataTypeStr=Inherit: Same as first input
  Multiply4 : Product  OutDataTypeStr=single
  Multiply5 : Product  Inputs=3
  Multiply6 : Product  OutDataTypeStr=single
  Sign{,1..6} (7 alike) : Signum
  Sqrt : Sqrt  SaturateOnIntegerOverflow=on
  Square : Math  Operator=square  SaturateOnIntegerOverflow=on
  Subtract{,1..5} (6 alike) : Sum  Inputs=+-  OutDataTypeStr=Inherit: Same as first input
  Subtract6 : Sum  Inputs=-+  OutDataTypeStr=Inherit: Same as first input
  const : Constant  Value=r0  OutDataTypeStr=single
  const1 : Constant  Value=h0  OutDataTypeStr=single
  fhan : Outport
  wires:
  v1/1 -> Add/1
  Sign/1 -> Multiply3/1
  Gain2/1 -> Multiply4/2  "sy"
  v2/1 -> Multiply1/1
  Gain3/1 -> Multiply5/3  "sa"
  Subtract/1 -> Gain1/1
  Subtract6/1 -> fhan/1
  Sign2/1 -> Subtract2/2
  Sign4/1 -> Subtract4/2
  Abs/1 -> Gain/1
  Add4/1 -> Multiply4/1
  Sign5/1 -> Subtract5/2
  Sqrt/1 -> Subtract/1  "a1"
  Subtract3/1 -> Sign4/1
  Add1/1 -> Multiply2/1
  Subtract1/1 -> Sign2/1
  Divide/1 -> Subtract5/1
  Multiply3/1 -> Add2/1
  Gain/1 -> Add1/2
  const/1 -> Multiply6/2, Gain4/1, Multiply/1
  Add3/1 -> Sign1/1
  Subtract5/1 -> Multiply5/2
  Multiply4/1 -> Add5/2
  const1/1 -> Multiply1/2, Square/1
  Add5/1 -> Sign6/1, Sign5/1, Divide/1, Subtract3/1, Add6/1  "a"
  Multiply1/1 -> Add4/3, Add2/2, Add/2  "a0"
  Add/1 -> Subtract1/1, Add3/1, Add4/2, Sign/1, Abs/1  "y"
  Subtract2/1 -> Gain2/1
  Add2/1 -> Add4/1, Add5/1  "a2"
  Subtract4/1 -> Gain3/1
  Gain4/1 -> Multiply5/1
  Multiply5/1 -> Subtract6/2
  Sign6/1 -> Multiply6/1
  Sign3/1 -> Subtract4/1
  Add6/1 -> Sign3/1
  Multiply/1 -> Subtract/2, Divide/2, Subtract3/2, Add6/2, Subtract1/2, Add3/2, Add1/1, Multiply2/2  "d"
  Multiply6/1 -> Subtract6/1
  Gain1/1 -> Multiply3/2
  Square/1 -> Multiply/2
  Multiply2/1 -> Sqrt/1
  Sign1/1 -> Subtract2/1

== system FMS/FMS Commander/Commander/Arm/MC_Mode/Assist/Position/Heading Command/Controller/Move Control/TD/fhan  ==
  v1 : Inport
  v2 : Inport  Port=2
  Abs : Abs
  Add{,1..3,5..6} (6 alike) : Sum  OutDataTypeStr=Inherit: Same as first input
  Add4 : Sum  Inputs=-++
  Divide : Product  Inputs=*/
  Gain : Gain  Gain=8
  Gain1 : Gain  Gain=0.5  OutDataTypeStr=Inherit: Same as input
  Gain2 : Gain  Gain=0.5  OutDataTypeStr=Inherit: Same as input
  Gain3 : Gain  Gain=0.5  OutDataTypeStr=Inherit: Same as input
  Gain4 : Gain  Gain=-1  OutDataTypeStr=Inherit: Same as input
  Multiply{,1..3} (4 alike) : Product  OutDataTypeStr=Inherit: Same as first input
  Multiply4 : Product  OutDataTypeStr=single
  Multiply5 : Product  Inputs=3
  Multiply6 : Product  OutDataTypeStr=single
  Sign{,1..6} (7 alike) : Signum
  Sqrt : Sqrt  SaturateOnIntegerOverflow=on
  Square : Math  Operator=square  SaturateOnIntegerOverflow=on
  Subtract{,1..5} (6 alike) : Sum  Inputs=+-  OutDataTypeStr=Inherit: Same as first input
  Subtract6 : Sum  Inputs=-+  OutDataTypeStr=Inherit: Same as first input
  const : Constant  Value=r0  OutDataTypeStr=single
  const1 : Constant  Value=h0  OutDataTypeStr=single
  fhan : Outport
  wires:
  v1/1 -> Add/1
  Sign/1 -> Multiply3/1
  Gain2/1 -> Multiply4/2  "sy"
  v2/1 -> Multiply1/1
  Gain3/1 -> Multiply5/3  "sa"
  Subtract/1 -> Gain1/1
  Subtract6/1 -> fhan/1
  Sign2/1 -> Subtract2/2
  Sign4/1 -> Subtract4/2
  Abs/1 -> Gain/1
  Add4/1 -> Multiply4/1
  Sign5/1 -> Subtract5/2
  Sqrt/1 -> Subtract/1  "a1"
  Subtract3/1 -> Sign4/1
  Add1/1 -> Multiply2/1
  Subtract1/1 -> Sign2/1
  Divide/1 -> Subtract5/1
  Multiply3/1 -> Add2/1
  Gain/1 -> Add1/2
  const/1 -> Multiply6/2, Gain4/1, Multiply/1
  Add3/1 -> Sign1/1
  Subtract5/1 -> Multiply5/2
  Multiply4/1 -> Add5/2
  const1/1 -> Multiply1/2, Square/1
  Add5/1 -> Sign6/1, Sign5/1, Divide/1, Subtract3/1, Add6/1  "a"
  Multiply1/1 -> Add4/3, Add2/2, Add/2  "a0"
  Add/1 -> Subtract1/1, Add3/1, Add4/2, Sign/1, Abs/1  "y"
  Subtract2/1 -> Gain2/1
  Add2/1 -> Add4/1, Add5/1  "a2"
  Subtract4/1 -> Gain3/1
  Gain4/1 -> Multiply5/1
  Multiply5/1 -> Subtract6/2
  Sign6/1 -> Multiply6/1
  Sign3/1 -> Subtract4/1
  Add6/1 -> Sign3/1
  Multiply/1 -> Subtract/2, Divide/2, Subtract3/2, Add6/2, Subtract1/2, Add3/2, Add1/1, Multiply2/2  "d"
  Multiply6/1 -> Subtract6/1
  Gain1/1 -> Multiply3/2
  Square/1 -> Multiply/2
  Multiply2/1 -> Sqrt/1
  Sign1/1 -> Subtract2/1

== system FMS/FMS Commander/Commander/Arm/MC_Mode/Assist/Position/Position Command/Controller/Move Control/TD/fhan  ==
  v1 : Inport
  v2 : Inport  Port=2
  Abs : Abs
  Add{,1..3,5..6} (6 alike) : Sum  OutDataTypeStr=Inherit: Same as first input
  Add4 : Sum  Inputs=-++
  Divide : Product  Inputs=*/
  Gain : Gain  Gain=8
  Gain1 : Gain  Gain=0.5  OutDataTypeStr=Inherit: Same as input
  Gain2 : Gain  Gain=0.5  OutDataTypeStr=Inherit: Same as input
  Gain3 : Gain  Gain=0.5  OutDataTypeStr=Inherit: Same as input
  Gain4 : Gain  Gain=-1  OutDataTypeStr=Inherit: Same as input
  Multiply{,1..3} (4 alike) : Product  OutDataTypeStr=Inherit: Same as first input
  Multiply4 : Product  OutDataTypeStr=single
  Multiply5 : Product  Inputs=3
  Multiply6 : Product  OutDataTypeStr=single
  Sign{,1..6} (7 alike) : Signum
  Sqrt : Sqrt  SaturateOnIntegerOverflow=on
  Square : Math  Operator=square  SaturateOnIntegerOverflow=on
  Subtract{,1..5} (6 alike) : Sum  Inputs=+-  OutDataTypeStr=Inherit: Same as first input
  Subtract6 : Sum  Inputs=-+  OutDataTypeStr=Inherit: Same as first input
  const : Constant  Value=r0  OutDataTypeStr=single
  const1 : Constant  Value=h0  OutDataTypeStr=single
  fhan : Outport
  wires:
  v1/1 -> Add/1
  Sign/1 -> Multiply3/1
  Gain2/1 -> Multiply4/2  "sy"
  v2/1 -> Multiply1/1
  Gain3/1 -> Multiply5/3  "sa"
  Subtract/1 -> Gain1/1
  Subtract6/1 -> fhan/1
  Sign2/1 -> Subtract2/2
  Sign4/1 -> Subtract4/2
  Abs/1 -> Gain/1
  Add4/1 -> Multiply4/1
  Sign5/1 -> Subtract5/2
  Sqrt/1 -> Subtract/1  "a1"
  Subtract3/1 -> Sign4/1
  Add1/1 -> Multiply2/1
  Subtract1/1 -> Sign2/1
  Divide/1 -> Subtract5/1
  Multiply3/1 -> Add2/1
  Gain/1 -> Add1/2
  const/1 -> Multiply6/2, Gain4/1, Multiply/1
  Add3/1 -> Sign1/1
  Subtract5/1 -> Multiply5/2
  Multiply4/1 -> Add5/2
  const1/1 -> Multiply1/2, Square/1
  Add5/1 -> Sign6/1, Sign5/1, Divide/1, Subtract3/1, Add6/1  "a"
  Multiply1/1 -> Add4/3, Add2/2, Add/2  "a0"
  Add/1 -> Subtract1/1, Add3/1, Add4/2, Sign/1, Abs/1  "y"
  Subtract2/1 -> Gain2/1
  Add2/1 -> Add4/1, Add5/1  "a2"
  Subtract4/1 -> Gain3/1
  Gain4/1 -> Multiply5/1
  Multiply5/1 -> Subtract6/2
  Sign6/1 -> Multiply6/1
  Sign3/1 -> Subtract4/1
  Add6/1 -> Sign3/1
  Multiply/1 -> Subtract/2, Divide/2, Subtract3/2, Add6/2, Subtract1/2, Add3/2, Add1/1, Multiply2/2  "d"
  Multiply6/1 -> Subtract6/1
  Gain1/1 -> Multiply3/2
  Square/1 -> Multiply/2
  Multiply2/1 -> Sqrt/1
  Sign1/1 -> Subtract2/1

== system FMS/FMS Commander/Commander/Arm/MC_Mode/Assist/Stabilize/Heading Command/Controller/Move Control/TD/fhan  ==
  v1 : Inport
  v2 : Inport  Port=2
  Abs : Abs
  Add{,1..3,5..6} (6 alike) : Sum  OutDataTypeStr=Inherit: Same as first input
  Add4 : Sum  Inputs=-++
  Divide : Product  Inputs=*/
  Gain : Gain  Gain=8
  Gain1 : Gain  Gain=0.5  OutDataTypeStr=Inherit: Same as input
  Gain2 : Gain  Gain=0.5  OutDataTypeStr=Inherit: Same as input
  Gain3 : Gain  Gain=0.5  OutDataTypeStr=Inherit: Same as input
  Gain4 : Gain  Gain=-1  OutDataTypeStr=Inherit: Same as input
  Multiply{,1..3} (4 alike) : Product  OutDataTypeStr=Inherit: Same as first input
  Multiply4 : Product  OutDataTypeStr=single
  Multiply5 : Product  Inputs=3
  Multiply6 : Product  OutDataTypeStr=single
  Sign{,1..6} (7 alike) : Signum
  Sqrt : Sqrt  SaturateOnIntegerOverflow=on
  Square : Math  Operator=square  SaturateOnIntegerOverflow=on
  Subtract{,1..5} (6 alike) : Sum  Inputs=+-  OutDataTypeStr=Inherit: Same as first input
  Subtract6 : Sum  Inputs=-+  OutDataTypeStr=Inherit: Same as first input
  const : Constant  Value=r0  OutDataTypeStr=single
  const1 : Constant  Value=h0  OutDataTypeStr=single
  fhan : Outport
  wires:
  v1/1 -> Add/1
  Sign/1 -> Multiply3/1
  Gain2/1 -> Multiply4/2  "sy"
  v2/1 -> Multiply1/1
  Gain3/1 -> Multiply5/3  "sa"
  Subtract/1 -> Gain1/1
  Subtract6/1 -> fhan/1
  Sign2/1 -> Subtract2/2
  Sign4/1 -> Subtract4/2
  Abs/1 -> Gain/1
  Add4/1 -> Multiply4/1
  Sign5/1 -> Subtract5/2
  Sqrt/1 -> Subtract/1  "a1"
  Subtract3/1 -> Sign4/1
  Add1/1 -> Multiply2/1
  Subtract1/1 -> Sign2/1
  Divide/1 -> Subtract5/1
  Multiply3/1 -> Add2/1
  Gain/1 -> Add1/2
  const/1 -> Multiply6/2, Gain4/1, Multiply/1
  Add3/1 -> Sign1/1
  Subtract5/1 -> Multiply5/2
  Multiply4/1 -> Add5/2
  const1/1 -> Multiply1/2, Square/1
  Add5/1 -> Sign6/1, Sign5/1, Divide/1, Subtract3/1, Add6/1  "a"
  Multiply1/1 -> Add4/3, Add2/2, Add/2  "a0"
  Add/1 -> Subtract1/1, Add3/1, Add4/2, Sign/1, Abs/1  "y"
  Subtract2/1 -> Gain2/1
  Add2/1 -> Add4/1, Add5/1  "a2"
  Subtract4/1 -> Gain3/1
  Gain4/1 -> Multiply5/1
  Multiply5/1 -> Subtract6/2
  Sign6/1 -> Multiply6/1
  Sign3/1 -> Subtract4/1
  Add6/1 -> Sign3/1
  Multiply/1 -> Subtract/2, Divide/2, Subtract3/2, Add6/2, Subtract1/2, Add3/2, Add1/1, Multiply2/2  "d"
  Multiply6/1 -> Subtract6/1
  Gain1/1 -> Multiply3/2
  Square/1 -> Multiply/2
  Multiply2/1 -> Sqrt/1
  Sign1/1 -> Subtract2/1

== system FMS/FMS Commander/Commander/Arm/MC_Mode/Auto/Mission/Mission_SubSystem/Heading Commander/Heading Control/Heading Control/Bus_Selection ==
  FMS_In : Inport
  Bus Selector2 : BusSelector  OutputSignals=INS_Out.psi
  psi_rad : Outport
  wires:
  Bus Selector2/1 -> psi_rad/1  "<psi>"
  FMS_In/1 -> Bus Selector2/1

== system FMS/FMS Commander/Commander/Arm/MC_Mode/Auto/Mission/Mission_SubSystem/Heading Commander/Heading Control/Heading Control/psi_saturation ==
  psi_in : Inport
  Abs : Abs
  Add : Sum  Inputs=-+
  Compare To Constant : simulink/Logic and Bit Operations/Compare To Constant  relop=>  const=pi  OutDataTypeStr=boolean
  Constant : Constant  Value=2*pi  OutDataTypeStr=single
  Constant1 : Constant  Value=2*pi  OutDataTypeStr=single
  Multiply : Product
  Rem : Math  Operator=rem  SaturateOnIntegerOverflow=on
  Sign : Signum
  Switch : Switch  Criteria=u2 > Threshold
  psi_rad : Outport
  wires:
  Constant1/1 -> Rem/2
  psi_in/1 -> Rem/1
  Switch/1 -> psi_rad/1
  Sign/1 -> Multiply/2
  Constant/1 -> Multiply/1
  Multiply/1 -> Add/1
  Add/1 -> Switch/1
  Compare To Constant/1 -> Switch/2
  Abs/1 -> Compare To Constant/1
  Rem/1 -> Abs/1, Switch/3, Add/2, Sign/1

== system FMS/FMS Commander/Commander/Arm/MC_Mode/Auto/Mission/Mission_SubSystem/Heading Commander/Heading Control/TD/fhan  ==
  v1 : Inport
  v2 : Inport  Port=2
  Abs : Abs
  Add{,1..3,5..6} (6 alike) : Sum  OutDataTypeStr=Inherit: Same as first input
  Add4 : Sum  Inputs=-++
  Divide : Product  Inputs=*/
  Gain : Gain  Gain=8
  Gain1 : Gain  Gain=0.5  OutDataTypeStr=Inherit: Same as input
  Gain2 : Gain  Gain=0.5  OutDataTypeStr=Inherit: Same as input
  Gain3 : Gain  Gain=0.5  OutDataTypeStr=Inherit: Same as input
  Gain4 : Gain  Gain=-1  OutDataTypeStr=Inherit: Same as input
  Multiply{,1..3} (4 alike) : Product  OutDataTypeStr=Inherit: Same as first input
  Multiply4 : Product  OutDataTypeStr=single
  Multiply5 : Product  Inputs=3
  Multiply6 : Product  OutDataTypeStr=single
  Sign{,1..6} (7 alike) : Signum
  Sqrt : Sqrt  SaturateOnIntegerOverflow=on
  Square : Math  Operator=square  SaturateOnIntegerOverflow=on
  Subtract{,1..5} (6 alike) : Sum  Inputs=+-  OutDataTypeStr=Inherit: Same as first input
  Subtract6 : Sum  Inputs=-+  OutDataTypeStr=Inherit: Same as first input
  const : Constant  Value=r0  OutDataTypeStr=single
  const1 : Constant  Value=h0  OutDataTypeStr=single
  fhan : Outport
  wires:
  Sign1/1 -> Subtract2/1
  Multiply2/1 -> Sqrt/1
  Square/1 -> Multiply/2
  Gain1/1 -> Multiply3/2
  Multiply6/1 -> Subtract6/1
  Multiply/1 -> Multiply2/2, Add1/1, Add3/2, Subtract1/2, Add6/2, Subtract3/2, Divide/2, Subtract/2  "d"
  Add6/1 -> Sign3/1
  Sign3/1 -> Subtract4/1
  Sign6/1 -> Multiply6/1
  Multiply5/1 -> Subtract6/2
  Gain4/1 -> Multiply5/1
  Subtract4/1 -> Gain3/1
  Add2/1 -> Add5/1, Add4/1  "a2"
  Subtract2/1 -> Gain2/1
  Add/1 -> Abs/1, Sign/1, Add4/2, Add3/1, Subtract1/1  "y"
  Multiply1/1 -> Add/2, Add2/2, Add4/3  "a0"
  Add5/1 -> Add6/1, Subtract3/1, Divide/1, Sign5/1, Sign6/1  "a"
  const1/1 -> Square/1, Multiply1/2
  Multiply4/1 -> Add5/2
  Subtract5/1 -> Multiply5/2
  Add3/1 -> Sign1/1
  const/1 -> Multiply/1, Gain4/1, Multiply6/2
  Gain/1 -> Add1/2
  Multiply3/1 -> Add2/1
  Divide/1 -> Subtract5/1
  Subtract1/1 -> Sign2/1
  Add1/1 -> Multiply2/1
  Subtract3/1 -> Sign4/1
  Sqrt/1 -> Subtract/1  "a1"
  Sign5/1 -> Subtract5/2
  Add4/1 -> Multiply4/1
  Abs/1 -> Gain/1
  Sign4/1 -> Subtract4/2
  Sign2/1 -> Subtract2/2
  Subtract6/1 -> fhan/1
  Subtract/1 -> Gain1/1
  Gain3/1 -> Multiply5/3  "sa"
  v2/1 -> Multiply1/1
  Gain2/1 -> Multiply4/2  "sy"
  Sign/1 -> Multiply3/1
  v1/1 -> Add/1

== system FMS/FMS Commander/Commander/Arm/MC_Mode/Auto/Mission/Mission_SubSystem/Velocity Commander/Hold Position/Altitude Hold/Controller ==
  motion_state : Inport
  In Bus Element : Inport  Port=2  PortName=FMS_In
  In Bus Element1 : Inport  Port=2  PortName=FMS_In
  Brake Control : Subsystem  TreatAsAtomicUnit=on
  Hold Control : Subsystem  TreatAsAtomicUnit=on
  Merge : Merge  Inputs=3
  Move Control : Subsystem  TreatAsAtomicUnit=on
  Saturation1 : Saturate  UpperLimit=FMS_PARAM.VEL_Z_LIM  LowerLimit=-FMS_PARAM.VEL_Z_LIM
  Switch Case : SwitchCase  CaseConditions={MotionState.Hold, MotionState.Brake, MotionState.Move}  ShowDefaultCase=off
  w_cmd_mPs : Outport
  wires:
  Move Control/1(w_cmd_mPs) -> Merge/3
  Brake Control/1(psi_rate_cmd_radPs) -> Merge/2
  Hold Control/1(w_cmd_mPs) -> Merge/1
  In Bus Element/1 -> Hold Control/1(FMS_In)
  Switch Case/3 -> Move Control/Action
  Switch Case/2 -> Brake Control/Action
  Switch Case/1 -> Hold Control/Action
  motion_state/1 -> Switch Case/1
  Saturation1/1 -> w_cmd_mPs/1
  Merge/1 -> Saturation1/1
  In Bus Element1/1 -> Move Control/1(FMS_In)
